simulink model "chaine_cod"  (R2026b)
settings: Solver=FixedStepDiscrete  StopTime=1000  FixedStep=1/(7*L)
values from neighbouring files (symbols this model uses):
  Ac = A*sqrt(4/7)    [partie4_teb.m]    (also in test_cod.m; test_retard.m)
  graine = round(P.graine)    [Parametres.m]    (also in Partie2.m = P.graine; parametres_perso.m = mod(sum(c .* (1:numel(c)) * 31) + 7 * numel(c), 2^31 - 1))
  L = P.L    [Parametres.m]    (also in construire_codeur.m = 'simulink/Logic and Bit Operations/Logical Operator'; construire_decodeur.m = 'simulink/Logic and Bit Operations/Logical Operator')
  seuil = 0    [test_cod.m]    (also in test_ech.m; test_gauss.m = seuils(k); test_retard.m; test_unif.m = seuils(k))
  sigma2 = A^2*L/(2*EbN0)    [test_cod.m]    (also in test_ech.m = A^2 * L / (2*EbN0); test_int.m = A^2 * L / (2*EbN0); test_retard.m)
libraries: simulink x1, dspstat3 x1, dspsigops x1
settings Model: Creator=INS NAWEL  LastModifiedBy=INS NAWEL

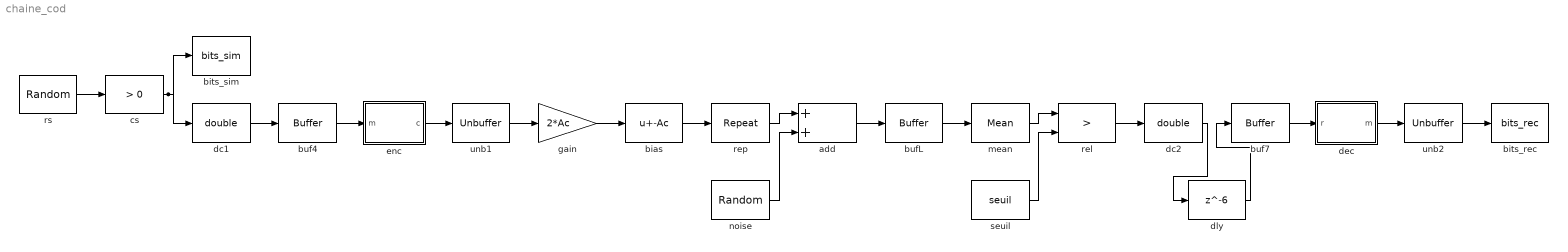
== system chaine_cod ==
  add : Sum
  bias : Bias  Bias=-Ac  SaturateOnIntegerOverflow=off
  bits_rec : ToWorkspace  VariableName=bits_rec  SampleTime=1
  bits_sim : ToWorkspace  VariableName=bits_sim  SampleTime=1
  buf4 : Buffer  N=4  OutputFrames=off
  buf7 : Buffer  N=7  OutputFrames=off
  bufL : Buffer  N=L  OutputFrames=off
  cs : simulink/Logic and Bit Operations/Compare To Constant  relop=>  const=0  OutDataTypeStr=boolean
  dc1 : DataTypeConversion  OutDataTypeStr=double  SaturateOnIntegerOverflow=off  RndMeth=Floor
  dc2 : DataTypeConversion  OutDataTypeStr=double  SaturateOnIntegerOverflow=off  RndMeth=Floor
  dec : MATLAB Function  TreatAsAtomicUnit=on
  dly : Delay  DelayLength=6
  enc : MATLAB Function  TreatAsAtomicUnit=on
  gain : Gain  Gain=2*Ac
  mean : dspstat3/Mean  run=off  InputProcessing=Columns as channels (frame based)  reset_popup=None  directionMode=Entire input  dimension=1  roiEnable=off  roiType=Rectangles  roiPortion=Entire ROI  roiOutput=Individual statistics for each ROI  roiFlag=off  roundingMode=Floor  overflowMode=off  outputDataTypeStr=Inherit: Same as accumulator  outputMin=[]  outputMax=[]  outputLastDataTypeStr=Inherit: Same as accumulator
  noise : RandomNumber  Variance=sigma2  Seed=graine+4  SampleTime=4/(7*L)
  rel : RelationalOperator  Operator=>  OutDataTypeStr=boolean  RndMeth=Simplest  InputSameDT=off
  rep : dspsigops/Repeat  FactorSource=Dialog parameter  N=L  Nmax=16  RateOptions=Allow multirate processing  ic=0  mode=Unused parameter value
      settings: LibrarySourceBlock=dsphdlsupportsigops/Repeat
  rs : RandomNumber  Seed=graine+1  SampleTime=1
  seuil : Constant  Value=seuil
  unb1 : Unbuffer
  unb2 : Unbuffer
  wires:
  rs/1 -> cs/1
  cs/1 -> bits_sim/1, dc1/1
  dc1/1 -> buf4/1
  buf4/1 -> enc/1(m)
  enc/1(c) -> unb1/1
  unb1/1 -> gain/1
  gain/1 -> bias/1
  bias/1 -> rep/1
  rep/1 -> add/1
  noise/1 -> add/2
  add/1 -> bufL/1
  bufL/1 -> mean/1
  mean/1 -> rel/1
  seuil/1 -> rel/2
  rel/1 -> dc2/1
  dc2/1 -> dly/1
  dly/1 -> buf7/1
  buf7/1 -> dec/1(r)
  dec/1(m) -> unb2/1
  unb2/1 -> bits_rec/1

== matlab function chaine_cod/enc ==
  data: m input; c output
function c = enc(m)
%#codegen
P = [1 1 0; 0 1 1; 1 1 1; 1 0 1];
G = [eye(4) P];
c = mod(G'*double(m(:)), 2);
end

== matlab function chaine_cod/dec ==
  data: r input; m output
function m = dec(r)
%#codegen
P = [1 1 0; 0 1 1; 1 1 1; 1 0 1];
H = [P' eye(3)];
x = double(r(:));
s = mod(H*x, 2);
idx = s(1) + 2*s(2) + 4*s(3);
pos = [5 6 1 7 4 2 3];
if idx > 0
    j = pos(idx);
    x(j) = 1 - x(j);
end
m = x(1:4);
end
